simulink model "DCHR_A51_TripDelay_2"  (R2026a)
settings: Solver=FixedStepDiscrete  StopTime=603900  FixedStep=900
settings Model: Creator=Lysda  LastModifiedBy=Lysda

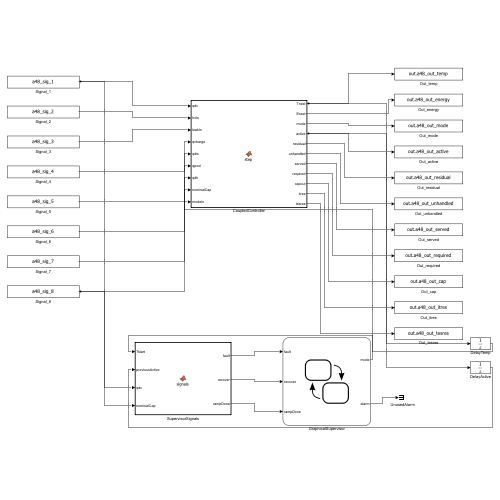
[thumbnail: Simulink's stored preview of the top-level diagram]
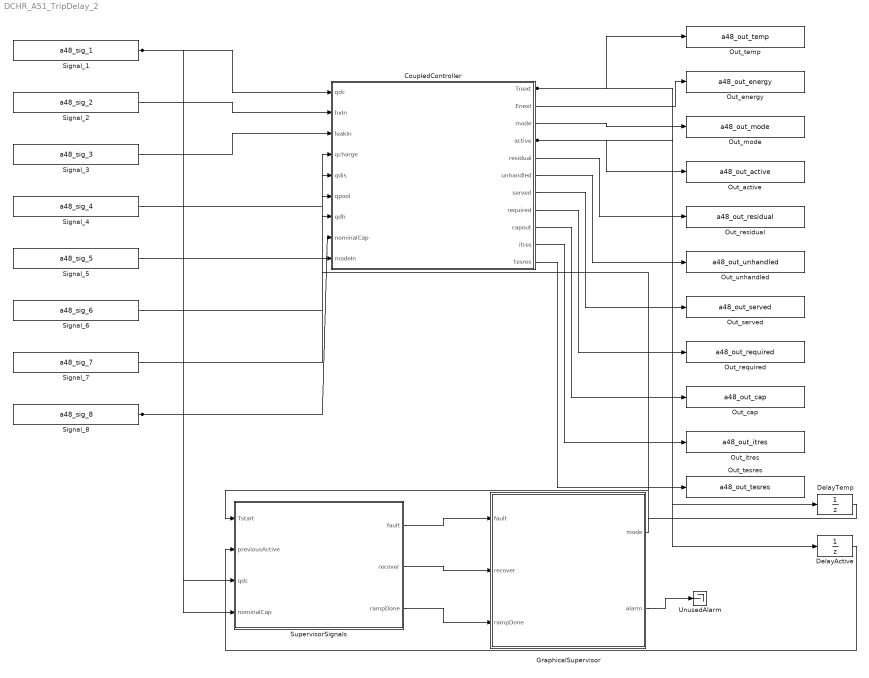
== system DCHR_A51_TripDelay_2 ==
  CoupledController : MATLAB Function  TreatAsAtomicUnit=on
  DelayActive : UnitDelay  SampleTime=900
  DelayTemp : UnitDelay  InitialCondition=30  SampleTime=900
  GraphicalSupervisor : Stateflow chart  TreatAsAtomicUnit=on
  Out_active : ToWorkspace  VariableName=a48_out_active  SampleTime=-1
  Out_cap : ToWorkspace  VariableName=a48_out_cap  SampleTime=-1
  Out_energy : ToWorkspace  VariableName=a48_out_energy  SampleTime=-1
  Out_itres : ToWorkspace  VariableName=a48_out_itres  SampleTime=-1
  Out_mode : ToWorkspace  VariableName=a48_out_mode  SampleTime=-1
  Out_required : ToWorkspace  VariableName=a48_out_required  SampleTime=-1
  Out_residual : ToWorkspace  VariableName=a48_out_residual  SampleTime=-1
  Out_served : ToWorkspace  VariableName=a48_out_served  SampleTime=-1
  Out_temp : ToWorkspace  VariableName=a48_out_temp  SampleTime=-1
  Out_tesres : ToWorkspace  VariableName=a48_out_tesres  SampleTime=-1
  Out_unhandled : ToWorkspace  VariableName=a48_out_unhandled  SampleTime=-1
  Signal_1 : FromWorkspace  VariableName=a48_sig_1
  Signal_2 : FromWorkspace  VariableName=a48_sig_2
  Signal_3 : FromWorkspace  VariableName=a48_sig_3
  Signal_4 : FromWorkspace  VariableName=a48_sig_4
  Signal_5 : FromWorkspace  VariableName=a48_sig_5
  Signal_6 : FromWorkspace  VariableName=a48_sig_6
  Signal_7 : FromWorkspace  VariableName=a48_sig_7
  Signal_8 : FromWorkspace  VariableName=a48_sig_8
  SupervisorSignals : MATLAB Function  TreatAsAtomicUnit=on
  UnusedAlarm : Terminator
  wires:
  Signal_1/1 -> CoupledController/1(qdc), SupervisorSignals/3(qdc)
  Signal_2/1 -> CoupledController/2(hxIn)
  Signal_3/1 -> CoupledController/3(leakIn)
  Signal_4/1 -> CoupledController/4(qcharge)
  Signal_5/1 -> CoupledController/5(qdis)
  Signal_6/1 -> CoupledController/6(qpool)
  Signal_7/1 -> CoupledController/7(qdh)
  Signal_8/1 -> CoupledController/8(nominalCap), SupervisorSignals/4(nominalCap)
  CoupledController/1(Tnext) -> Out_temp/1, DelayTemp/1
  CoupledController/2(Enext) -> Out_energy/1
  CoupledController/3(mode) -> Out_mode/1
  CoupledController/4(active) -> Out_active/1, DelayActive/1
  CoupledController/5(residual) -> Out_residual/1
  CoupledController/6(unhandled) -> Out_unhandled/1
  CoupledController/7(served) -> Out_served/1
  CoupledController/8(required) -> Out_required/1
  CoupledController/9(capout) -> Out_cap/1
  CoupledController/10(itres) -> Out_itres/1
  CoupledController/11(tesres) -> Out_tesres/1
  DelayTemp/1 -> SupervisorSignals/1(Tstart)
  DelayActive/1 -> SupervisorSignals/2(previousActive)
  SupervisorSignals/1(fault) -> GraphicalSupervisor/1(fault)
  SupervisorSignals/2(recover) -> GraphicalSupervisor/2(recover)
  SupervisorSignals/3(rampDone) -> GraphicalSupervisor/3(rampDone)
  GraphicalSupervisor/1(mode) -> CoupledController/9(modeIn)
  GraphicalSupervisor/2(alarm) -> UnusedAlarm/1

== matlab function DCHR_A51_TripDelay_2/SupervisorSignals ==
  data: Tstart input; fault output; previousActive input; qdc input; nominalCap input; recover output; rampDone output
function [fault,recover,rampDone] = signals(Tstart,previousActive,qdc,nominalCap)
%#codegen
fault=(nominalCap<=0 || Tstart>=42);
recover=(nominalCap>0 && Tstart<36);
rampDone=(previousActive+15000>=qdc-1e-8);
end

== matlab function DCHR_A51_TripDelay_2/CoupledController ==
  data: qdc input; Tnext output; hxIn input; leakIn input; qcharge input; qdis input; qpool input; qdh input; nominalCap input; modeIn input; Enext output; mode output; active output; residual output; unhandled output; served output; required output; capout output; itres output; tesres output
function [Tnext,Enext,mode,active,residual,unhandled,served,required,capout,itres,tesres] = step(qdc,hxIn,leakIn,qcharge,qdis,qpool,qdh,nominalCap,modeIn)
%#codegen
persistent E T prevActive prevShed prevMode res lastTrip effCap hpAvailable
if isempty(E)
 E=450*3.6e6;T=30;prevActive=0;prevShed=0;prevMode=0;res=0;lastTrip=false;effCap=330000;hpAvailable=0;
end
dt=900;Emax=900*3.6e6;
effCap=min(nominalCap,effCap+60000);
state=modeIn;
if state==1
 active=qdc;
elseif state==2
 active=0;
elseif state==3
 active=min(qdc,prevActive+15000);
elseif prevMode==3
 active=qdc;
else
 h0=min(hxIn,qdc);l0=min(leakIn,max(0,qdc-h0));
 av0=max(0,qdc-h0-l0);
 demand=qpool+qdh;loss0=.002*E/86400;
 dcap0=max(0,(E-dt*loss0)*.91/dt);
 dis0=min([qdis,demand,dcap0]);
 room0=max(0,(Emax-E+dt*(dis0/.91+loss0))/(dt*.93));
 charge0=min(qcharge,room0);
 need0=max(0,demand-dis0);desired0=need0+charge0;
 cop0=max(2,min(5,3.5+.04*(T-30)));
 source0=min(av0,desired0*(cop0-1)/cop0);
 required0=max(0,qdc-h0-l0-source0);
 target=min(.4*qdc,max(0,required0-effCap));
 shed=min(target,prevShed+15000);
 active=qdc-shed;
end
if state==2 && ~lastTrip
 res=.12*prevActive;
elseif res>0
 res=res*exp(-dt/3600);
end
active=min(active,max(0,qdc-res));
qit=active+res;
hx=min(hxIn,qit);leak=min(leakIn,max(0,qit-hx));
available=max(0,qit-hx-leak);
demand=qpool+qdh;loss=.002*E/86400;
discap=max(0,(E-dt*loss)*.91/dt);
dis=min([qdis,demand,discap]);
room=max(0,(Emax-E+dt*(dis/.91+loss))/(dt*.93));
creq=min(qcharge,room);need=max(0,demand-dis);
desired=need+creq;cop=max(2,min(5,3.5+.04*(T-30)));
sourceTarget=min(available,desired*(cop-1)/cop);
hpAvailable=hpAvailable+(1-exp(-dt/1800))*(sourceTarget-hpAvailable);
source=min(sourceTarget,hpAvailable);
power=source/(cop-1);cond=source+power;
servedhp=min(need,cond);charge=min(creq,max(0,cond-servedhp));
served=dis+servedhp;
Enext=max(0,min(Emax,E+dt*(.93*charge-dis/.91-loss)));
required=max(0,qit-hx-leak-source);
rejected=min(required,effCap);
unhandled=max(0,required-rejected);
passive=2000*max(0,T-30);
Tnext=max(30,T+dt*(unhandled-passive)/8e6);
itres=qit-hx-leak-source-rejected-unhandled;
tesres=Enext-E-dt*(.93*charge-dis/.91-loss);
mode=state;residual=res;capout=effCap;
E=Enext;T=Tnext;prevActive=active;prevShed=qdc-active;prevMode=state;lastTrip=(state==2);
end

== stateflow chart DCHR_A51_TripDelay_2/GraphicalSupervisor ==
  state ACTIVE
    entry: mode=0; alarm=0;
  state TRIP_PENDING
    entry: mode=1; alarm=1; pending=1;
    during: pending=pending+1;
  state RAMPING
    entry: mode=3; alarm=1;
  state TRIPPED
    entry: mode=2; alarm=2; good=0;
    during: if recover && ~fault; good=good+1; else; good=0; end
  TRIP_PENDING -> ACTIVE [order 1] : [~fault && recover]
  (default) -> ACTIVE
  RAMPING -> ACTIVE [order 1] : [rampDone && ~fault]
  RAMPING -> TRIP_PENDING [order 2] : [fault]
  ACTIVE -> TRIP_PENDING : [fault]
  TRIP_PENDING -> TRIPPED [order 2] : [pending>=2]
  TRIPPED -> RAMPING : [good>=1 && recover && ~fault]
  data: fault input; recover input; rampDone input; mode output; alarm output; pending local; good local
